simulink model "sm_motor_model"  (R2026b)
settings: Solver=ode4  StopTime=T  FixedStep=dt
values from neighbouring files (symbols this model uses):
  S = sim_param(q, D(k).ac, kp)    [deney_4a.m]    (also in dogrula_2.m = sim_param(q, h.ac, ref.kp); dogrula_3.m = sim_param(q, h.ac, kp); dogrula_b2.m = sim_param(q, ac, kp); dogrula_b2_dt.m = sim_param(q, ac, kp))
  Ts = t(2) - t(1)    [km_kestir.m]    (also in tani_Fs.m; tani_JM.m; tani_JM_kol.m; tani_Ks.m)
undefined symbols (not defined in the file or in its folder): Tsur
libraries: fl_lib x13, nesl_utility x9, ee_lib x1
settings Model: Creator=safak  LastModifiedBy=safak
settings DataIOCC: Decimation=dec  SaveTime=off  SignalLogging=off
settings DebuggingCC: AlgebraicLoopMsg=none
settings SimscapeCC: SimscapeLogType=all  SimscapeNominalValues="[{\"value\":\"1\",\"unit\":\"A\"},{\"value\":\"1\",\"unit\":\"bar\"},{\"value\":\"1\",\"unit\":\"cm^2\"},{\"value\":\"1\",\"unit\":\"cm^3/s\"},{\"value\":\"1\",\"unit\":\"kJ/kg\"},{\"value\":\"1\",\"unit\":\"kW\"},{\"value\":\"1\",\"unit\":\"l\"},{\"value\":\"1\",\"unit\":\"N\"},{\"value\":\"1\",\"unit\":\"N*m\"},{\"value\":\"1\",\"unit\":\"V\"},{\"value\":\"0.001\",\"unit\":\"Wb\"}]"  SimscapeUseEnergyAccounting=off

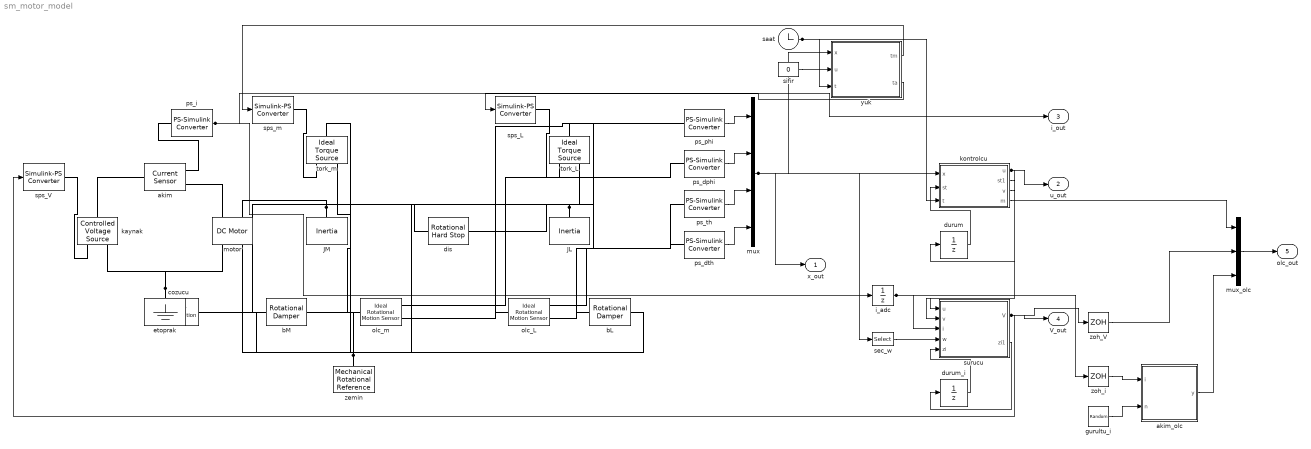
== system sm_motor_model ==
  JL : fl_lib/Mechanical/Rotational Elements/Inertia  inertia=S.JL kg*m^2  num_ports=foundation.enum.numPorts2.one  w_specify=on  w_priority=High  w=S.x0(4) rad/s  w_nominal_specify=off  w_nominal_value=1  w_nominal_unit=rad/s  t_specify=off  t_priority=None  t=0 N*m  t_nominal_specify=off  t_nominal_value=1  t_nominal_unit=N*m
  JM : fl_lib/Mechanical/Rotational Elements/Inertia  inertia=S.JM kg*m^2  num_ports=foundation.enum.numPorts2.one  w_specify=on  w_priority=High  w=S.x0(2) rad/s  w_nominal_specify=off  w_nominal_value=1  w_nominal_unit=rad/s  t_specify=off  t_priority=None  t=0 N*m  t_nominal_specify=off  t_nominal_value=1  t_nominal_unit=N*m
  akim : fl_lib/Electrical/Electrical Sensors/Current Sensor
  akim_olc : MATLAB Function  TreatAsAtomicUnit=on
  bL : fl_lib/Mechanical/Rotational Elements/Rotational Damper  D=S.bL N*m*s/rad  w_specify=off  w_priority=None  w=0 rad/s  w_nominal_specify=off  w_nominal_value=1  w_nominal_unit=rad/s  t_specify=off  t_priority=None  t=0 N*m  t_nominal_specify=off  t_nominal_value=1  t_nominal_unit=N*m
  bM : fl_lib/Mechanical/Rotational Elements/Rotational Damper  D=S.bM N*m*s/rad  w_specify=off  w_priority=None  w=0 rad/s  w_nominal_specify=off  w_nominal_value=1  w_nominal_unit=rad/s  t_specify=off  t_priority=None  t=0 N*m  t_nominal_specify=off  t_nominal_value=1  t_nominal_unit=N*m
  cozucu : nesl_utility/Solver Configuration  PhysicalDomain=network_engine_domain  SubClassName=solver  LeftPortType=input  RightPortType=generic  Tones=[]  Harmonics=[]  SimulateNoise=off  Profile=off  UseLocalSampling=off  EnableSwitchedLinearOptims=on  FrequencyDomain=off  UseCCode=off  RelTol=0.001  AbsTol=0.001  MinStep=1e-09  ToWorkspace=off  RevertToSquareIcSolve=off  NumHomotopyIterations=100  PhasorMode=off  PhasorModeNumHarmonics=1  ConsistencySolver=NEWTON_XTOL_AFTER_FTOL  CanonicalOrdering=CANONICAL  OptimizeIntermediates=OPTIMIZED  MulticoreSolverChoice=BACKWARD_EULER  IndexReductionMethod=DerivativeReplacement  DoDC=off  ResidualTolerance=1e-09  ConsistencyTolSource=GLOBAL  ConsistencyAbsTol=0.001  ConsistencyRelTol=0.001  ConsistencyTolFactor=0.001  UseLocalSolver=off  LocalSolverChoice=NE_BACKWARD_EULER_ADVANCER  ResolveIndetEquations=on  FunctionEvalNumThread=1  LocalSolverSampleTime=0.001  DoFixedCost=off  MaxNonlinIter=3  MaxModeIter=2  ComputeImpulses=off  ImpulseIterations=2  LinearAlgebra=auto  LinearAlgebraNumThread=0  EquationFormulation=NE_TIME_EF  DelaysMemoryBudget=1024  AutomaticFiltering=on  FilteringTimeConstant=0.001  PartitionStorageMethod=AS_NEEDED  PartitionMemoryBudget=1024  PartitionMethod=BALANCED  MultibodyUseLocalSolver=off  MultibodyLocalSolverChoice=ODE1  MultibodyLocalSolverSampleTime=0.001
  dis : fl_lib/Mechanical/Rotational Elements/Rotational Hard Stop  upper_bnd=S.r - (S.x0(1) - S.x0(3)) rad  lower_bnd=-S.r - (S.x0(1) - S.x0(3)) rad  model=simscape.enum.hardstop.smooth  stiff_up=S.Ks N*m/rad  stiff_low=S.Ks N*m/rad  D_up=S.cs N*m*s/rad  D_low=S.cs N*m*s/rad  transition=gecis rad  coeff_rest=0.7  w_tol=0.1 rad/s  trq_tol=0.001 N*m  w_specify=off  w_priority=None  w=0 rad/s  w_nominal_specify=off  w_nominal_value=1  w_nominal_unit=rad/s  t_specify=off  t_priority=None  t=0 N*m  t_nominal_specify=off  t_nominal_value=1  t_nominal_unit=N*m  phi_specify=off  phi_priority=High  phi=0 rad  phi_nominal_specify=off  phi_nominal_value=1  phi_nominal_unit=rad  M_specify=off  M_priority=None  M=0
  durum : UnitDelay  InitialCondition=S.st0  SampleTime=Ts
  durum_i : UnitDelay  SampleTime=Tsur
  etoprak : fl_lib/Electrical/Electrical Elements/Electrical Reference
  gurultu_i : RandomNumber  Seed=S.iSeed  SampleTime=Ts
  i_adc : UnitDelay  SampleTime=Tsur
  kaynak : fl_lib/Electrical/Electrical Sources/Controlled Voltage Source
  kontrolcu : MATLAB Function  TreatAsAtomicUnit=on
  motor : ee_lib/Electromechanical/Brushed Motors/DC Motor  field_option=ee.enum.field_option.pm  Rf=100 Ohm  Lf=1 H  Laf=0.15 H  If0=0 A  parameterization=ee.enum.dcparam_option.circuit_param  Ra=S.Ra Ohm  La=S.La H  emf_or_torque=ee.enum.emf_or_torque.kv  Kv=S.Km V*s/rad  Ki=6.876e-4 N*m/A  T_stall=0.24e-3 N*m  w_max=19100 rpm  w_rated=15000 rpm  P_rated=0.08 W  V_rated=1.5 V  lam_param=ee.enum.lam_param.damping  i_noload=0 A  V_i_noload=1.5 V  J=0 cm^2*g  lam=0 N*m*s/rad  speed0=0 rpm  alpha=3.93e-3 1/K  Tmeas=25 degC  thermal_mass=100 J/K  initial_temperature=25 degC
  mux : Mux
  mux_olc : Mux  Inputs=3
  olc_L : fl_lib/Mechanical/Mechanical Sensors/Ideal Rotational Motion Sensor  reference=foundation.enum.MeasurementReference.absolute  acceleration_port=false  velocity_port=true  position_port=true  wrap_angle=false  offset=S.x0(3) rad
  olc_m : fl_lib/Mechanical/Mechanical Sensors/Ideal Rotational Motion Sensor  reference=foundation.enum.MeasurementReference.absolute  acceleration_port=false  velocity_port=true  position_port=true  wrap_angle=false  offset=S.x0(1) rad
  ps_dphi : nesl_utility/PS-Simulink Converter  PhysicalDomain=network_engine_domain  SubClassName=ps_output  LeftPortType=input  RightPortType=output  PseudoPeriodic=off  Frequencies=[]  VectorFormat=inherit  Unit=rad/s  AffineConversion=off
  ps_dth : nesl_utility/PS-Simulink Converter  PhysicalDomain=network_engine_domain  SubClassName=ps_output  LeftPortType=input  RightPortType=output  PseudoPeriodic=off  Frequencies=[]  VectorFormat=inherit  Unit=rad/s  AffineConversion=off
  ps_i : nesl_utility/PS-Simulink Converter  PhysicalDomain=network_engine_domain  SubClassName=ps_output  LeftPortType=input  RightPortType=output  PseudoPeriodic=off  Frequencies=[]  VectorFormat=inherit  Unit=A  AffineConversion=off
  ps_phi : nesl_utility/PS-Simulink Converter  PhysicalDomain=network_engine_domain  SubClassName=ps_output  LeftPortType=input  RightPortType=output  PseudoPeriodic=off  Frequencies=[]  VectorFormat=inherit  Unit=rad  AffineConversion=off
  ps_th : nesl_utility/PS-Simulink Converter  PhysicalDomain=network_engine_domain  SubClassName=ps_output  LeftPortType=input  RightPortType=output  PseudoPeriodic=off  Frequencies=[]  VectorFormat=inherit  Unit=rad  AffineConversion=off
  saat : Clock
  sec_w : Selector  InputPortWidth=4  IndexOptions=Index vector (dialog)  Indices=2  OutputSizes=1
  sifir : Constant  Value=0
  sps_L : nesl_utility/Simulink-PS Converter  PhysicalDomain=network_engine_domain  SubClassName=ps_input  LeftPortType=input  RightPortType=output  PseudoPeriodic=off  Frequencies=[]  NoiseDistribution=none  NoiseParameters=[]  Unit=N*m  AffineConversion=off  FilteringAndDerivatives=provide  SimscapeFilterOrder=1  InputFilterTimeConstant=0.001  UdotUserProvided=0
  sps_V : nesl_utility/Simulink-PS Converter  PhysicalDomain=network_engine_domain  SubClassName=ps_input  LeftPortType=input  RightPortType=output  PseudoPeriodic=off  Frequencies=[]  NoiseDistribution=none  NoiseParameters=[]  Unit=V  AffineConversion=off  FilteringAndDerivatives=zero  SimscapeFilterOrder=1  InputFilterTimeConstant=0.001  UdotUserProvided=0
  sps_m : nesl_utility/Simulink-PS Converter  PhysicalDomain=network_engine_domain  SubClassName=ps_input  LeftPortType=input  RightPortType=output  PseudoPeriodic=off  Frequencies=[]  NoiseDistribution=none  NoiseParameters=[]  Unit=N*m  AffineConversion=off  FilteringAndDerivatives=provide  SimscapeFilterOrder=1  InputFilterTimeConstant=0.001  UdotUserProvided=0
  surucu : MATLAB Function  TreatAsAtomicUnit=on
  tork_L : fl_lib/Mechanical/Mechanical Sources/Ideal Torque Source
  tork_m : fl_lib/Mechanical/Mechanical Sources/Ideal Torque Source
  yuk : MATLAB Function  TreatAsAtomicUnit=on
  zemin : fl_lib/Mechanical/Rotational Elements/Mechanical Rotational Reference
  zoh_V : ZeroOrderHold  SampleTime=Ts
  zoh_i : ZeroOrderHold  SampleTime=Ts
  x_out : Outport
  u_out : Outport  Port=2
  i_out : Outport  Port=3
  V_out : Outport  Port=4
  olc_out : Outport  Port=5
  wires:
  ps_phi/1 -> mux/1
  ps_dphi/1 -> mux/2
  ps_th/1 -> mux/3
  ps_dth/1 -> mux/4
  mux/1 -> yuk/1(x), kontrolcu/1(x), x_out/1, sec_w/1
  sifir/1 -> yuk/2(u)
  saat/1 -> yuk/3(t), kontrolcu/3(t)
  yuk/1(tm) -> sps_m/1
  yuk/2(ta) -> sps_L/1
  durum/1 -> kontrolcu/2(st)
  kontrolcu/2(st1) -> durum/1
  kontrolcu/1(u) -> u_out/1, surucu/1(u)
  kontrolcu/3(v) -> surucu/2(v)
  ps_i/1 -> i_adc/1, i_out/1
  i_adc/1 -> surucu/3(i), zoh_i/1
  sec_w/1 -> surucu/4(w)
  durum_i/1 -> surucu/5(zi)
  surucu/2(zi1) -> durum_i/1
  surucu/1(V) -> sps_V/1, V_out/1, zoh_V/1
  zoh_i/1 -> akim_olc/1(i)
  gurultu_i/1 -> akim_olc/2(n)
  kontrolcu/4(m) -> mux_olc/1
  zoh_V/1 -> mux_olc/2
  akim_olc/1(y) -> mux_olc/3
  mux_olc/1 -> olc_out/1
  connections:
  cozucu/RConn1 -- bM/RConn1 -- bL/RConn1 -- tork_m/RConn2 -- tork_L/RConn2 -- zemin/LConn1 -- motor/RConn2
  dis/LConn1 -- JM/LConn1 -- bM/LConn1 -- tork_m/LConn1 -- olc_m/LConn1 -- motor/LConn2
  dis/RConn1 -- bL/LConn1 -- tork_L/LConn1 -- JL/LConn1 -- olc_L/LConn1
  sps_m/RConn1 -- tork_m/RConn1
  sps_L/RConn1 -- tork_L/RConn1
  olc_m/RConn2 -- ps_phi/LConn1
  olc_m/RConn1 -- ps_dphi/LConn1
  olc_L/RConn2 -- ps_th/LConn1
  olc_L/RConn1 -- ps_dth/LConn1
  kaynak/LConn1 -- akim/LConn1
  akim/RConn2 -- motor/LConn1
  etoprak/LConn1 -- motor/RConn1 -- kaynak/RConn2
  sps_V/RConn1 -- kaynak/RConn1
  akim/RConn1 -- ps_i/LConn1

== matlab function sm_motor_model/kontrolcu ==
  settings: updateMethod=DISCRETE  sampleTime=Ts
  data: x input; u output; st input; t input; st1 output; v output; m output; S parameter
function [u, st1, v, m] = ayrik(x, st, t, S)
% m: firmware'in Ts'de kaydedeceği ölçümler [th_L (AS5600, gecikmeli); phi (enkoder); v (kestirim); u]
% v: kontrolcünün kullandığı hız (sürücünün zıt EMK kompanzasyonu için dışarı verilir)
% Sensör + kontrolcü, durumsuz yazım (Simscape modeli için). blok_sensor + blok_kontrolcu ile aynı hesap;
% durumlar persistent yerine dışarıdaki Unit Delay'de tutulur: st = [tampon(21); vhat; yprev; z].
% Böylece Simscape ağının (Hard Stop yüzünden) yapısal cebirsel döngüsünü Simulink çözebilir.
%
% Deney kaynağı (firmware'in üreteceği sinyal, Ts örneklemeli; sim_param'daki S.dny_*):
%   S.dny_yer = 0  yok (kontrolcü olduğu gibi)
%               1  referansa eklenir:      e = ref + d - thm          (kapalı çevrim konum uyarımı)
%               2  tork komutuna eklenir:  u0 = kontrolcü + d          (kapalı çevrim tork enjeksiyonu)
%               3  açık çevrim:            u0 = dny_u0 + d, kontrolcü kapalı, integral donuk
%   d = dny_A * şekil(t - dny_t0), yalnız dny_t0 <= t < dny_t0 + dny_Td:
%     S.dny_sek = 1 dikdörtgen (basamak; kısa Td ile darbe), 2 doğrusal chirp f0 -> f1,
%                 3 logaritmik chirp f0 -> f1, 4 sinüs (sabit f0)
%   Serbest salınım: dny_yer = 3, dny_A = 0, dny_u0 = 0 ve başlangıç sapması (p.adim / p.x0).
%
% Hız kestirimi (S.hiz; fv = Inf ise hepsi yerine gerçek hız):
%   0 fark      (y_k - y_{k-1})/Ts + birinci dereceden alçak geçiren (kesim fv)        [varsayılan]
%   1 periyot   son iki enkoder kenarı arasındaki süre: v = n q / (t_kenar - t_önceki_kenar).
%               Kenar zamanı donanımda GPIO kesmesi + µs sayaçla damgalanır; burada iki örnek arasında
%               gerçek açının doğrusal aradeğerlemesiyle bulunur. Yön değişince v = 0. Kenar gelmezse
%               |v| <= q / (t - t_son_kenar) (yavaşlayınca sıfıra iner). Filtre yok.
%   2 gozlemci  ikinci dereceden izleme gözlemcisi (Euler, Ts): e = y - th_hat,
%               th_hat += Ts (w_hat + 2 wo e), w_hat += Ts wo^2 e, wo = 2 pi fv (kritik sönümlü)
% Ek durumlar st(25:28): periyot [phi_önceki (gerçek), t_son_kenar, yön, v]; gozlemci [th_hat, w_hat, 0, 0].
buf = st(1:21);  vhat = st(22);  yprev = st(23);  z = st(24);  ek = st(25:28);
vi = 3;  qv = S.qL;
if S.motorD > 0, vi = 1;  qv = S.qM; end
% --- sensör ---
thm = olc(x(3), S.qL);
if S.gL > 0
    buf = [buf(2:end); thm];
    thm = buf(21 - S.gL);
end
if S.fv_inf > 0
    v = x(vi + 1);
elseif S.hiz == 1
    [v, ek] = periyot(x(vi), t, ek, qv, S.Ts);
    yprev = olc(x(vi), qv);
elseif S.hiz == 2
    yv = olc(x(vi), qv);
    wo = 2*pi*S.fv;
    e_o = yv - ek(1);
    ek(1) = ek(1) + S.Ts*(ek(2) + 2*wo*e_o);
    ek(2) = ek(2) + S.Ts*wo^2*e_o;
    v = ek(2);
    yprev = yv;
else
    yv = olc(x(vi), qv);
    vhat = vhat + S.aV*((yv - yprev)/S.Ts - vhat);
    yprev = yv;
    v = vhat;
end
% --- deney kaynağı ---
d = 0;
if S.dny_yer > 0, d = kaynak(t, S); end
% --- kontrolcü ---
e = S.ref - thm;
if S.dny_yer == 1, e = e + d; end
if S.ppi > 0
    ev = S.kp*e - v;
    u0 = S.KV*ev + S.KI*z;
    iz = ev;
else
    u0 = S.Kp*e + S.Ki*z - S.Kd*v;
    iz = e;
end
if S.dny_yer == 2, u0 = u0 + d; end
acik = S.dny_yer == 3;
if acik, u0 = S.dny_u0 + d; end
u = min(max(u0, -S.Tmax), S.Tmax);
doy = (u0 > S.Tmax && iz > 0) || (u0 < -S.Tmax && iz < 0);
if ~doy && ~acik, z = z + iz*S.Ts; end
if abs(u) < S.olu, u = 0; end
st1 = [buf; vhat; yprev; z; ek];
m = [thm; olc(x(1), S.qM); v; u];   % firmware kaydı: AS5600 (gecikmeli), enkoder, hız kestirimi, tork komutu
end

function [v, ek] = periyot(phi, t, ek, q, Ts)
% ek = [phi_önceki, t_son_kenar, yön, v]. t_son_kenar < 0: henüz kenar yok.
phip = ek(1);  tl = ek(2);  yon = ek(3);  v = ek(4);
n1 = floor(phi/q);  n0 = floor(phip/q);
if n1 ~= n0
    d = sign(n1 - n0);
    if d > 0, sev = n1*q; else, sev = (n1 + 1)*q; end         % son geçilen kenar
    a = (sev - phip)/(phi - phip);  a = min(max(a, 0), 1);
    te = t - Ts + a*Ts;                                        % kenar zamanı (aradeğerleme)
    if d == yon && tl >= 0 && te > tl
        v = d*abs(n1 - n0)*q/(te - tl);
    else
        v = 0;                                                 % ilk kenar ya da yön değişimi
    end
    tl = te;  yon = d;
elseif tl >= 0 && t > tl
    vs = q/(t - tl);                                           % kenar gelmedikçe hız sınırı düşer
    if abs(v) > vs, v = sign(v)*vs; end
end
ek = [phi; tl; yon; v];
end

function y = olc(x, q)
y = x;
if q > 0, y = q*floor(x/q); end
end

function d = kaynak(t, S)
d = 0;
tau = t - S.dny_t0;
if tau < 0 || tau >= S.dny_Td, return; end
switch S.dny_sek
    case 1
        s = 1;
    case 2      % anlık frekans f0 + (f1 - f0) tau / Td
        s = sin(2*pi*(S.dny_f0*tau + (S.dny_f1 - S.dny_f0)*tau^2/(2*S.dny_Td)));
    case 3      % anlık frekans f0 (f1/f0)^(tau/Td)
        k = log(S.dny_f1/S.dny_f0)/S.dny_Td;
        s = sin(2*pi*S.dny_f0*(exp(k*tau) - 1)/k);
    otherwise
        s = sin(2*pi*S.dny_f0*tau);
end
d = S.dny_A*s;
end

== matlab function sm_motor_model/yuk ==
  data: x input; u input; tm output; t input; ta output; S parameter
function [tm, ta] = yuk(x, u, t, S)
% Simscape modelinde fiziksel ağa verilen torklar (Simulink tarafında hesaplanır):
%   tm: motor eylemsizliğine etkiyen net tork = kontrolcü torku - Stribeck sürtünmesi
%   ta: kola etkiyen dış tork = yerçekimi + yük bozucusu
% Viskoz sürtünmeler (bM, bL) ve dişli teması Simscape bloklarındadır.
dphi = x(2);  th = x(3);
tf = 0;
if S.Fc > 0
    tf = (S.Fc + (S.Fs - S.Fc)*exp(-(dphi/S.vs)^2)) * tanh(dphi/S.veps);
end
tm = u - tf;
bz = 0;
if t >= S.d0 && t < S.dT
    bz = S.dA*sin(2*pi*S.df*(t - S.d0));
end
ta = -S.mgl*sin(th) + bz;
end

== matlab function sm_motor_model/surucu ==
  settings: updateMethod=DISCRETE  sampleTime=Tsur
  data: u input; V output; v input; i input; w input; zi input; zi1 output; S parameter
function [V, zi1] = surucu(u, v, i, w, zi, S)
% Firmware'in tork komutunu (u) motor gerilimine çevirmesi + DRV8874 (ortalama model, PWM anahtarlaması yok).
% Örnekleme Tsur (akım döngüsü / PWM güncelleme hızı). Durumsuz yazım: akım PI integrali zi dışarıda (Unit Delay).
%   S.mot = 1  gerilim modu:            V = Ra u / Km               (zıt EMK sönümü devrede)
%   S.mot = 2  zıt EMK kompanzasyonu:   V = Ra u / Km + Km v        (v: kontrolcünün kullandığı motor hızı)
%   S.mot = 3  akım döngüsü:            i_ref = u / Km (sınırlı), PI (IPROPI ölçümü, Tsur hızında)
%              i girişi bir Tsur gecikmeli gelir (ADC örneği -> hesap -> PWM; sm_model_kur'daki i_adc)
% Donanım: besleme +-Vs ile doyum; DRV8874 akım sınırı Ilim (kıyıcı akımı Ilim'de tutar; ortalama
% modelde gerilim, kararlı akımı Ilim'i aşmayacak şekilde sınırlanır: |V - Km w| <= Ra Ilim).
% Km, Ra, Ilim kol tarafına indirgenmiş eşdeğer motor büyüklükleridir (sim_param).
zi1 = zi;  e = 0;
if S.mot == 3
    iref = min(max(u/S.Km, -S.Ilim), S.Ilim);
    e = iref - i;
    Vc = S.Kpi*e + zi;
elseif S.mot == 2
    Vc = S.Ra*u/S.Km + S.Km*v;
else
    Vc = S.Ra*u/S.Km;
end
V = min(max(Vc, S.Km*w - S.Ra*S.Ilim), S.Km*w + S.Ra*S.Ilim);   % akım sınırı
V = min(max(V, -S.Vs), S.Vs);                                    % besleme
if S.mot == 3
    if V == Vc || (V < Vc && e < 0) || (V > Vc && e > 0)         % anti-windup
        zi1 = zi + S.Kii*S.Tsur*e;
    end
end
end

== matlab function sm_motor_model/akim_olc ==
  settings: updateMethod=DISCRETE  sampleTime=Ts
  data: i input; y output; n input; S parameter
function y = akim(i, n, S)
% IPROPI akım ölçümü, firmware kaydı (Ts örneklemeli): ADC gürültüsü + nicemleme.
%   i: ADC'nin gördüğü akım (i_adc, bir Tsur gecikmeli), n: birim varyanslı gürültü (Random Number bloğu)
%   S.iGur: gürültü std [A], S.qI: ADC basamağı akım cinsinden [A] (0 = ideal)
y = i + S.iGur*n;
if S.qI > 0, y = S.qI*round(y/S.qI); end
end
